simulink model "FMT_PIDAllocationProbe"  (R2026b)
settings: Solver=FixedStepDiscrete  StopTime=0.01  FixedStep=0.001
undefined symbols (not defined in the file): RateDcutoff, RateIlimit, RateKaw, RateKd, RateKi, RateKp
settings Model: DataDictionary=Flight_Parameters.sldd  Creator=26718  LastModifiedBy=26718

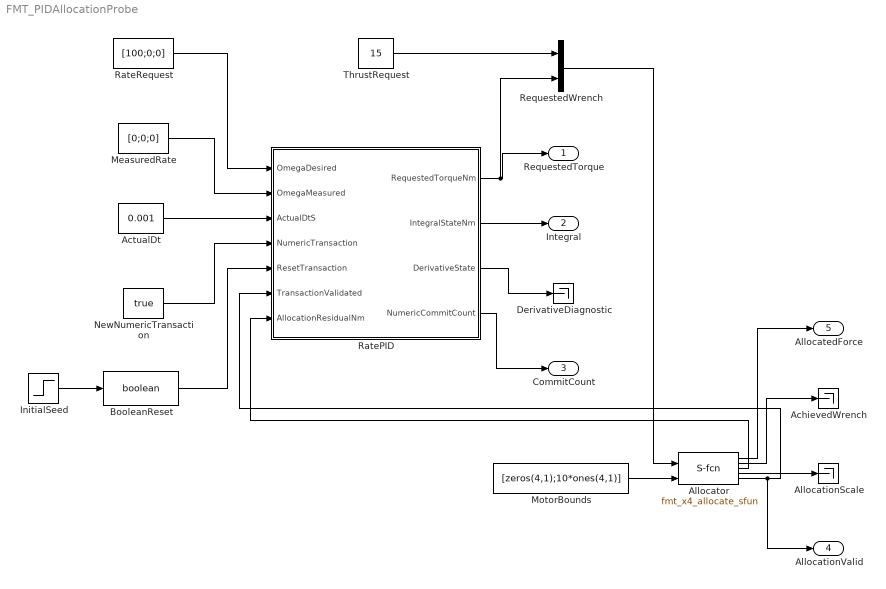
== system FMT_PIDAllocationProbe ==
  AchievedWrench : Terminator
  ActualDt : Constant  Value=0.001
  AllocationScale : Terminator
  Allocator : S-Function  FunctionName=fmt_x4_allocate_sfun  Parameters=AllocationMatrices  SFunctionDeploymentMode=off  EnableBusSupport=off
  BooleanReset : DataTypeConversion  OutDataTypeStr=boolean  SaturateOnIntegerOverflow=off  RndMeth=Floor
  DerivativeDiagnostic : Terminator
  InitialSeed : Step  Time=0.001  InitialValue=1  FinalValue=0  SampleTime=0.001
  MeasuredRate : Constant  Value=[0;0;0]
  MotorBounds : Constant  Value=[zeros(4,1);10*ones(4,1)]
  NewNumericTransaction : Constant  Value=true  OutDataTypeStr=boolean
  RatePID : Subsystem
  RateRequest : Constant  Value=[100;0;0]
  RequestedWrench : Mux  Inputs=2
  ThrustRequest : Constant  Value=15
  RequestedTorque : Outport
  Integral : Outport  Port=2
  CommitCount : Outport  Port=3
  AllocationValid : Outport  Port=4
  AllocatedForce : Outport  Port=5
  wires:
  Allocator/4 -> AllocationScale/1
  Allocator/2 -> AchievedWrench/1
  Allocator/1 -> AllocatedForce/1
  RatePID/4(NumericCommitCount) -> CommitCount/1
  RatePID/3(DerivativeState) -> DerivativeDiagnostic/1
  RatePID/2(IntegralStateNm) -> Integral/1
  MotorBounds/1 -> Allocator/2
  RequestedWrench/1 -> Allocator/1
  RatePID/1(RequestedTorqueNm) -> RequestedWrench/2, RequestedTorque/1
  ThrustRequest/1 -> RequestedWrench/1
  Allocator/3 -> RatePID/7(AllocationResidualNm)
  Allocator/5 -> RatePID/6(TransactionValidated), AllocationValid/1
  BooleanReset/1 -> RatePID/5(ResetTransaction)
  InitialSeed/1 -> BooleanReset/1
  NewNumericTransaction/1 -> RatePID/4(NumericTransaction)
  ActualDt/1 -> RatePID/3(ActualDtS)
  MeasuredRate/1 -> RatePID/2(OmegaMeasured)
  RateRequest/1 -> RatePID/1(OmegaDesired)

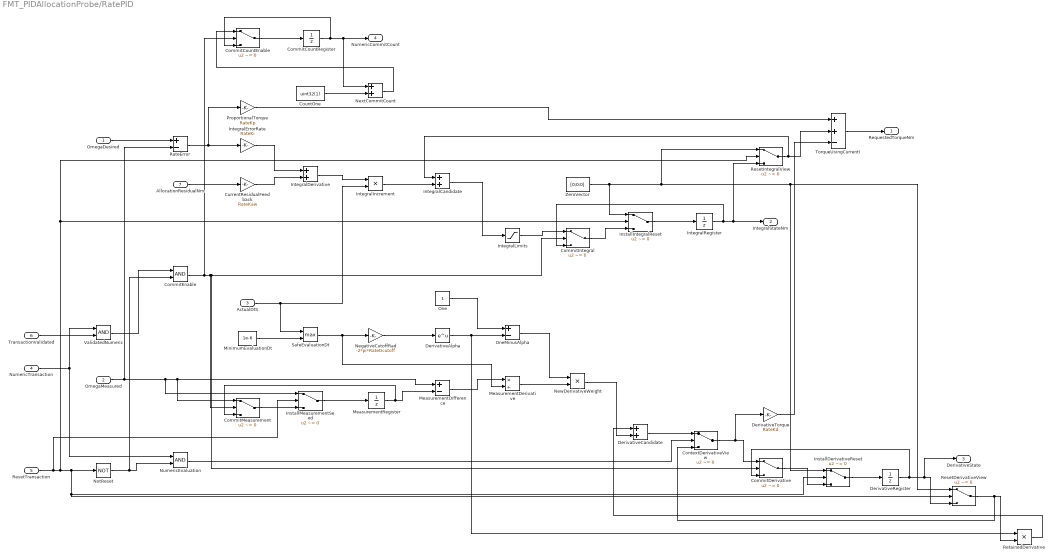
== system FMT_PIDAllocationProbe/RatePID ==
  OmegaDesired : Inport  OutDataTypeStr=double  PortDimensions=3
  OmegaMeasured : Inport  Port=2  OutDataTypeStr=double  PortDimensions=3
  ActualDtS : Inport  Port=3  OutDataTypeStr=double  PortDimensions=1
  NumericTransaction : Inport  Port=4  OutDataTypeStr=boolean  PortDimensions=1
  ResetTransaction : Inport  Port=5  OutDataTypeStr=boolean  PortDimensions=1
  TransactionValidated : Inport  Port=6  OutDataTypeStr=boolean  PortDimensions=1
  AllocationResidualNm : Inport  Port=7  OutDataTypeStr=double  PortDimensions=3
  CommitCountEnable : Switch  Criteria=u2 ~= 0  SaturateOnIntegerOverflow=off  InputSameDT=off
  CommitCountRegister : UnitDelay  InitialCondition=uint32(0)  SampleTime=-1
  CommitDerivative : Switch  Criteria=u2 ~= 0  SaturateOnIntegerOverflow=off  InputSameDT=off
  CommitEnable : Logic  IconShape=distinctive  AllPortsSameDT=off  OutDataTypeStr=boolean
  CommitIntegral : Switch  Criteria=u2 ~= 0  SaturateOnIntegerOverflow=off  InputSameDT=off
  CommitMeasurement : Switch  Criteria=u2 ~= 0  SaturateOnIntegerOverflow=off  InputSameDT=off
  ContextDerivativeView : Switch  Criteria=u2 ~= 0  SaturateOnIntegerOverflow=off  InputSameDT=off
  CountOne : Constant  Value=uint32(1)  OutDataTypeStr=uint32
  CurrentResidualFeedback : Gain  Gain=RateKaw
  DerivativeAlpha : Math
  DerivativeCandidate : Sum
  DerivativeRegister : UnitDelay  InitialCondition=[0;0;0]  SampleTime=-1
  DerivativeTorque : Gain  Gain=RateKd
  InstallDerivativeReset : Switch  Criteria=u2 ~= 0  SaturateOnIntegerOverflow=off  InputSameDT=off
  InstallIntegralReset : Switch  Criteria=u2 ~= 0  SaturateOnIntegerOverflow=off  InputSameDT=off
  InstallMeasurementSeed : Switch  Criteria=u2 ~= 0  SaturateOnIntegerOverflow=off  InputSameDT=off
  IntegralCandidate : Sum
  IntegralDerivative : Sum
  IntegralErrorRate : Gain  Gain=RateKi
  IntegralIncrement : Product  Inputs=**
  IntegralLimits : Saturate  UpperLimit=RateIlimit  LowerLimit=-RateIlimit
  IntegralRegister : UnitDelay  InitialCondition=[0;0;0]  SampleTime=-1
  MeasurementDerivative : Product  Inputs=*/
  MeasurementDifference : Sum  Inputs=+-
  MeasurementRegister : UnitDelay  InitialCondition=[0;0;0]  SampleTime=-1
  MinimumEvaluationDt : Constant  Value=1e-6
  NegativeCutoffRad : Gain  Gain=-2*pi*RateDcutoff
  NewDerivativeWeight : Product  Inputs=**
  NextCommitCount : Sum  OutDataTypeStr=uint32
  NotReset : Logic  Operator=NOT  IconShape=distinctive  AllPortsSameDT=off  OutDataTypeStr=boolean
  NumericEvaluation : Logic  IconShape=distinctive  AllPortsSameDT=off  OutDataTypeStr=boolean
  One : Constant
  OneMinusAlpha : Sum  Inputs=+-
  ProportionalTorque : Gain  Gain=RateKp
  RateError : Sum  Inputs=+-
  ResetDerivativeView : Switch  Criteria=u2 ~= 0  SaturateOnIntegerOverflow=off  InputSameDT=off
  ResetIntegralView : Switch  Criteria=u2 ~= 0  SaturateOnIntegerOverflow=off  InputSameDT=off
  RetainedDerivative : Product  Inputs=**
  SafeEvaluationDt : MinMax  Function=max  Inputs=2
  TorqueUsingCurrentI : Sum  Inputs=++-
  ValidatedNumeric : Logic  IconShape=distinctive  AllPortsSameDT=off  OutDataTypeStr=boolean
  ZeroVector : Constant  Value=[0;0;0]
  RequestedTorqueNm : Outport
  IntegralStateNm : Outport  Port=2
  DerivativeState : Outport  Port=3
  NumericCommitCount : Outport  Port=4
  wires:
  CommitCountEnable/1 -> CommitCountRegister/1
  NextCommitCount/1 -> CommitCountEnable/1
  CountOne/1 -> NextCommitCount/2
  CommitCountRegister/1 -> NextCommitCount/1, NumericCommitCount/1, CommitCountEnable/3
  InstallMeasurementSeed/1 -> MeasurementRegister/1
  CommitMeasurement/1 -> InstallMeasurementSeed/3
  InstallDerivativeReset/1 -> DerivativeRegister/1
  CommitDerivative/1 -> InstallDerivativeReset/3
  InstallIntegralReset/1 -> IntegralRegister/1
  CommitIntegral/1 -> InstallIntegralReset/3
  CommitEnable/1 -> CommitIntegral/2, CommitDerivative/2, CommitMeasurement/2, CommitCountEnable/2
  IntegralLimits/1 -> CommitIntegral/1
  NotReset/1 -> CommitEnable/2, NumericEvaluation/2
  ValidatedNumeric/1 -> CommitEnable/1
  TransactionValidated/1 -> ValidatedNumeric/2
  NumericTransaction/1 -> ValidatedNumeric/1, NumericEvaluation/1
  IntegralCandidate/1 -> IntegralLimits/1
  IntegralIncrement/1 -> IntegralCandidate/2
  IntegralDerivative/1 -> IntegralIncrement/1
  CurrentResidualFeedback/1 -> IntegralDerivative/2
  IntegralErrorRate/1 -> IntegralDerivative/1
  AllocationResidualNm/1 -> CurrentResidualFeedback/1
  TorqueUsingCurrentI/1 -> RequestedTorqueNm/1
  DerivativeTorque/1 -> TorqueUsingCurrentI/3
  ResetIntegralView/1 -> TorqueUsingCurrentI/2, IntegralCandidate/1
  ProportionalTorque/1 -> TorqueUsingCurrentI/1
  ContextDerivativeView/1 -> DerivativeTorque/1, CommitDerivative/1
  NumericEvaluation/1 -> ContextDerivativeView/2
  DerivativeCandidate/1 -> ContextDerivativeView/1
  NewDerivativeWeight/1 -> DerivativeCandidate/2
  RetainedDerivative/1 -> DerivativeCandidate/1
  MeasurementDerivative/1 -> NewDerivativeWeight/2
  OneMinusAlpha/1 -> NewDerivativeWeight/1
  ResetDerivativeView/1 -> RetainedDerivative/2, ContextDerivativeView/3
  DerivativeAlpha/1 -> OneMinusAlpha/2, RetainedDerivative/1
  One/1 -> OneMinusAlpha/1
  NegativeCutoffRad/1 -> DerivativeAlpha/1
  SafeEvaluationDt/1 -> MeasurementDerivative/2, NegativeCutoffRad/1
  MeasurementDifference/1 -> MeasurementDerivative/1
  MeasurementRegister/1 -> MeasurementDifference/2, CommitMeasurement/3
  DerivativeRegister/1 -> DerivativeState/1, ResetDerivativeView/3, CommitDerivative/3
  IntegralRegister/1 -> IntegralStateNm/1, ResetIntegralView/3, CommitIntegral/3
  ResetTransaction/1 -> ResetDerivativeView/2, InstallDerivativeReset/2, NotReset/1, ResetIntegralView/2, InstallIntegralReset/2, InstallMeasurementSeed/2
  ZeroVector/1 -> ResetDerivativeView/1, InstallDerivativeReset/1, ResetIntegralView/1, InstallIntegralReset/1
  MinimumEvaluationDt/1 -> SafeEvaluationDt/2
  ActualDtS/1 -> SafeEvaluationDt/1, IntegralIncrement/2
  RateError/1 -> ProportionalTorque/1, IntegralErrorRate/1
  OmegaMeasured/1 -> MeasurementDifference/1, CommitMeasurement/1, InstallMeasurementSeed/1, RateError/2
  OmegaDesired/1 -> RateError/1
